simulink model "LHS_Robot"  (R2026a)
settings: Solver=FixedStepAuto  StopTime=2.72
values from neighbouring files (symbols this model uses):
  b = 4.50    (= 4.5)    [run_simulation.m]    (also in sim_dashboard.m = prs(j,2))
  c_L = 1.5813    [run_simulation.m]
  E_max = 6.6    [run_simulation.m]
  K = 0.002811691    [run_simulation.m]
  Ki = 2.5    [run_simulation.m]
  Kp = 0.18    [run_simulation.m]
  m_L = 1.1763    [run_simulation.m]
  mass = 0.85    [run_simulation.m]
  N = numel(tracks)    [route_planner.m]    (also in run_simulation.m = 48; sim_dashboard.m = size(starts, 1))
  R_wheel = 0.065/2    (= 0.0325)    [run_simulation.m]
  Ra = 7.953487304    [run_simulation.m]
  Ts = 0.02    [run_simulation.m]
  Ts_fast = 2e-5    (= 2e-05)    [run_simulation.m]
libraries: slpidlib x1
settings Model: DataDictionary=Robot.sldd  Creator=AdrianStark  LastModifiedBy=AdrianStark
settings ModelReferenceCC: ModelReferenceMinAlgLoopOccurrences=on

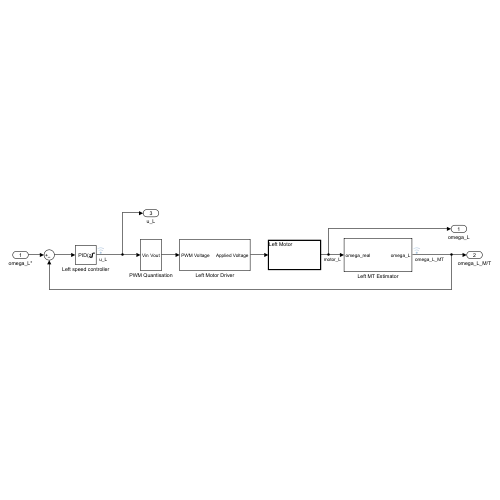
[thumbnail: Simulink's stored preview of the top-level diagram]
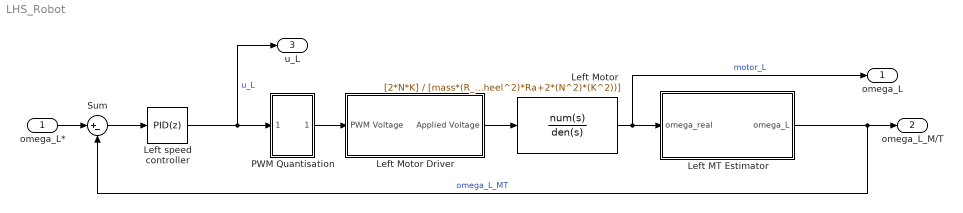
== system LHS_Robot ==
  omega_L* : Inport  OutDataTypeStr=double  PortDimensions=1  SampleTime=[0,1]
  Left MT Estimator : Subsystem
  Left Motor : TransferFcn  Numerator=[2*N*K]  Denominator=[mass*(R_wheel^2)*Ra (b*(R_wheel^2)*Ra+2*(N^2)*(K^2))]
  Left Motor Driver : Subsystem
  Left speed controller : slpidlib/PID Controller  Controller=PID  Form=Parallel  TimeDomain=Discrete-time  UseExternalTs=off  SampleTime=Ts  IntegratorMethod=Trapezoidal  FilterMethod=Forward Euler  ControllerParametersSource=internal  P=Kp  I=Ki  UseKiTs=off  D=0  UseExternalDerivativeSource=off  N=100  UseFilter=on  TunerSelectOption=Transfer Function Based (PID Tuner App)  InitialConditionSource=internal  InitialConditionForIntegrator=0  InitialConditionForFilter=0  DifferentiatorICPrevScaledInput=0  ExternalReset=none  TrackingMode=off  Kt=1  LimitOutput=on  SatLimitsSource=internal  UpperSaturationLimit=E_max  LowerSaturationLimit=0  LinearizeAsGain=on  AntiWindupMode=clamping  Kb=1  LimitIntegrator=off  UpperIntegratorSaturationLimit=inf  LowerIntegratorSaturationLimit=-inf  POutMin=[]  POutMax=[]  IOutMin=[]  IOutMax=[]  DOutMin=[]  DOutMax=[]  NOutMin=[]  NOutMax=[]  SumOutMin=[]  SumOutMax=[]  SaturationOutMin=[]  SaturationOutMax=[]  PParamMin=[]  PParamMax=[]  IParamMin=[]  IParamMax=[]  DParamMin=[]  DParamMax=[]  NParamMin=[]  NParamMax=[]  KbParamMin=[]  KbParamMax=[]  KtParamMin=[]  KtParamMax=[]  KbOutMin=[]  KbOutMax=[]  KtOutMin=[]  KtOutMax=[]  IntegratorOutMin=[]  IntegratorOutMax=[]  FilterOutMin=[]  FilterOutMax=[]  SumI1OutMin=[]  SumI1OutMax=[]  SumI2OutMin=[]  SumI2OutMax=[]  SumI3OutMin=[]  SumI3OutMax=[]  SumI4OutMin=[]  SumI4OutMax=[]  SumDOutMin=[]  SumDOutMax=[]  DifferentiatorOutMin=[]  DifferentiatorOutMax=[]  FilterDiffOutCoefMin=[]  FilterDiffOutCoefMax=[]  ReciprocalOutMin=[]  ReciprocalOutMax=[]  SumDenOutMin=[]  SumDenOutMax=[]  SumNumOutMin=[]  SumNumOutMax=[]  DivideOutMin=[]  DivideOutMax=[]  UdiffTsProdOutMin=[]  UdiffTsProdOutMax=[]  NTsProdOutMin=[]  NTsProdOutMax=[]  UintegralTsProdOutMin=[]  UintegralTsProdOutMax=[]  UngainTsProdOutMin=[]  UngainTsProdOutMax=[]  ClampingZeroOutDataTypeStr=Inherit: Inherit via back propagation  ClampingZeroOutMin=[]  ClampingZeroOutMax=[]  FilterDenConstantOutDataTypeStr=Inherit: Inherit via back propagation  FilterDenConstantOutMin=[]  FilterDenConstantOutMax=[]  PCopyOutDataTypeStr=Inherit: Inherit via back propagation  PCopyOutMin=[]  PCopyOutMax=[]  NCopyOutDataTypeStr=Inherit: Inherit via back propagation  NCopyOutMin=[]  NCopyOutMax=[]  IntegratorContinuousStateAttributes=''  IntegratorStateMustResolveToSignalObject=off  IntegratorRTWStateStorageClass=Auto  FilterContinuousStateAttributes=''  FilterStateMustResolveToSignalObject=off  FilterRTWStateStorageClass=Auto  ParallelPVariant=InternalParameters  IdealPVariant=Disabled  IVariant=InternalParameters  DVariant=InternalParameters  IntegratorVariant=Discrete  SatVariant=Enabled  AWVariant=DiscClampingParallel  PCopyVariant=Disabled  TRVariant=Disabled  FdbkBlocksVariant=Feedback  IdealPFdbkVariant=Passthrough  SatFdbkVariant=Passthrough  DerivativeFilterVariant=ForwardEulerFilter  NVariant=InternalParameters  NCopyVariant=Disabled  FilterICVariant=InternalICsFilter  IntegratorICVariant=InternalICs  ExternalResetVariant=Disabled  TRSumVariant=Passthrough  SumFdbkVariant=Enabled  SumVariant=Sum_PID  TsampFilterVariant=InternalTs  TsampNgainVariant=Passthrough  TsampIntegralVariant=Disabled_SignalSpec  ExternalSaturationOutDataTypeStr=Inherit: Same as second input  DerivativeSourceVariant=ErrorSignal  PreIntVariant=InternalPreInt
  PWM Quantisation : Subsystem
  Sum : Sum  Inputs=|+-
  omega_L : Outport
  omega_L_M/T : Outport  Port=2  OutDataTypeStr=double  PortDimensions=1  SampleTime=[0.02,0]
  u_L : Outport  Port=3
  wires:
  Left Motor/1 -> omega_L/1, Left MT Estimator/1(omega_real)  "motor_L"
  Left MT Estimator/1(omega_L) -> omega_L_M/T/1, Sum/2  "omega_L_MT"
  omega_L*/1 -> Sum/1
  Sum/1 -> Left speed controller/1
  Left speed controller/1 -> u_L/1, PWM Quantisation/1(Vin)  "u_L"
  Left Motor Driver/1(Applied Voltage) -> Left Motor/1
  PWM Quantisation/1(Vout) -> Left Motor Driver/1(PWM Voltage)

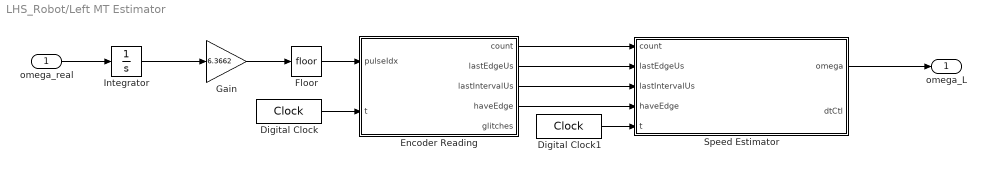
== system LHS_Robot/Left MT Estimator ==
  omega_real : Inport
  Digital Clock : DigitalClock  SampleTime=Ts_fast
  Digital Clock1 : DigitalClock  SampleTime=Ts
  Encoder Reading : MATLAB Function  TreatAsAtomicUnit=on  SystemSampleTime=Ts_fast
  Floor : Rounding
  Gain : Gain  Gain=6.3662
  Integrator : Integrator
  Speed Estimator : MATLAB Function  TreatAsAtomicUnit=on  SystemSampleTime=Ts
  omega_L : Outport
  wires:
  omega_real/1 -> Integrator/1
  Encoder Reading/3(lastIntervalUs) -> Speed Estimator/3(lastIntervalUs)
  Encoder Reading/1(count) -> Speed Estimator/1(count)
  Floor/1 -> Encoder Reading/1(pulseIdx)
  Integrator/1 -> Gain/1
  Speed Estimator/1(omega) -> omega_L/1
  Gain/1 -> Floor/1
  Encoder Reading/4(haveEdge) -> Speed Estimator/4(haveEdge)
  Digital Clock/1 -> Encoder Reading/2(t)
  Encoder Reading/2(lastEdgeUs) -> Speed Estimator/2(lastEdgeUs)
  Digital Clock1/1 -> Speed Estimator/5(t)

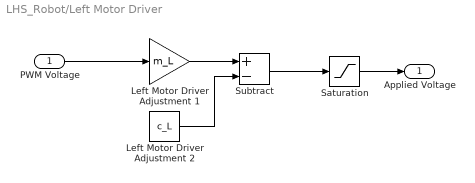
== system LHS_Robot/Left Motor Driver ==
  PWM Voltage : Inport
  Left Motor Driver Adjustment 1 : Gain  Gain=m_L
  Left Motor Driver Adjustment 2 : Constant  Value=c_L
  Saturation : Saturate  UpperLimit=6.6  LowerLimit=0
  Subtract : Sum  Inputs=+-
  Applied Voltage : Outport
  wires:
  Saturation/1 -> Applied Voltage/1
  Left Motor Driver Adjustment 2/1 -> Subtract/2
  PWM Voltage/1 -> Left Motor Driver Adjustment 1/1
  Subtract/1 -> Saturation/1
  Left Motor Driver Adjustment 1/1 -> Subtract/1

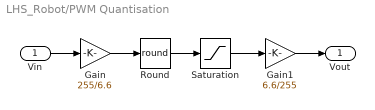
== system LHS_Robot/PWM Quantisation ==
  Vin : Inport
  Gain : Gain  Gain=255/6.6
  Gain1 : Gain  Gain=6.6/255
  Round : Rounding  Operator=round
  Saturation : Saturate  UpperLimit=255  LowerLimit=0
  Vout : Outport
  wires:
  Gain1/1 -> Vout/1
  Vin/1 -> Gain/1
  Saturation/1 -> Gain1/1
  Round/1 -> Saturation/1
  Gain/1 -> Round/1

== matlab function LHS_Robot/Left MT Estimator/Speed Estimator ==
  data: count input; lastEdgeUs input; lastIntervalUs input; haveEdge input; omega output; t input; dtCtl output
function [omega, dtCtl] = mtTickEstimator(count, lastEdgeUs, lastIntervalUs, haveEdge, t)
%MTTICKESTIMATOR  Simulink model of the per-tick estimator in loop().
%
%   One instance per wheel. MATLAB Function block, Sample time = 0.020
%   (TICK_MS). Inputs come from encoderISR through a Rate Transition.
%
%   Reproduces, in order:
%     1. the ring buffer snapshot of (count, lastEdgeUs)
%     2. M/T over the LONGEST valid span, not just the full gate
%     3. the T fallback (one interval, reciprocated, decaying as 1/t)
%     4. the staleness ceiling and the stall timeout
%     5. the measured, clamped dt handed to the PID
%
%   dtCtl is constant at 0.020 in simulation because the model has no
%   serial writes to delay a tick. Leave the clamp in anyway - it costs
%   nothing and it documents what the firmware does.

%#codegen

% ---- Constants, matching the sketch -----------------------------------
WINDOW_TICKS     = 3;
NRING            = WINDOW_TICKS + 1;             % 4 slots, 60 ms max span
PULSES_PER_REV   = 40;                           % 20 slots x 2 edges x gear 1.0
RAD_PER_PULSE    = 2*pi/PULSES_PER_REV;          % 0.157080 rad
STALL_TIMEOUT_US = uint32(500000);
TICK_MS          = 20;
DT_MIN_S         = TICK_MS*0.0005;               % 0.010 s
DT_MAX_S         = TICK_MS*0.0040;               % 0.080 s

persistent ringCount ringEdge head fill lastCtlUs ctlPrimed
if isempty(head)
    ringCount = zeros(1, NRING, 'uint32');
    ringEdge  = zeros(1, NRING, 'uint32');
    head      = 0;                               % 0-based, as in C
    fill      = 0;
    lastCtlUs = uint32(0);
    ctlPrimed = false;
end

nowUs = uint32(t*1e6);

% ---- Snapshot into the ring -------------------------------------------
head = mod(head + 1, NRING);
ringCount(head+1) = count;
ringEdge(head+1)  = lastEdgeUs;
if fill <= WINDOW_TICKS
    fill = fill + 1;
end

omega  = 0;
haveMT = false;

% ---- M/T over the longest valid span ----------------------------------
% Search from the OLDEST usable snapshot forward, break on the first hit,
% so the span grows as history accumulates rather than jumping when the
% gate fills.
if fill >= 2
    startBack = fill - 1;
else
    startBack = 0;
end

for back = startBack:-1:1
    idx = mod(head + NRING - back, NRING);       % 0-based, as in C
    if ringCount(idx+1) < 1
        continue                                  % no edge existed yet
    end
    if count <= ringCount(idx+1)
        continue                                  % no new pulse since
    end
    dtEdgeUs = lastEdgeUs - ringEdge(idx+1);
    if dtEdgeUs == 0
        continue
    end
    omega  = double(count - ringCount(idx+1)) * RAD_PER_PULSE * 1e6 / double(dtEdgeUs);
    haveMT = true;
    break
end

% ---- T fallback --------------------------------------------------------
if ~haveMT && haveEdge && lastIntervalUs > 0
    sinceUs = nowUs - lastEdgeUs;
    if sinceUs < STALL_TIMEOUT_US
        if sinceUs > lastIntervalUs
            effUs = sinceUs;
        else
            effUs = lastIntervalUs;
        end
        omega = RAD_PER_PULSE * 1e6 / double(effUs);
    end
end

% ---- Staleness ceiling -------------------------------------------------
% The M/T window ends at the LAST EDGE, not at now, so without this a
% stopped wheel keeps re-reporting the speed from before it stopped.
if haveEdge
    sinceUs = nowUs - lastEdgeUs;
    if sinceUs >= STALL_TIMEOUT_US
        omega = 0;
    elseif sinceUs > 0
        bound = RAD_PER_PULSE * 1e6 / double(sinceUs);
        if omega > bound
            omega = bound;
        end
    end
end

% ---- Measured control interval ----------------------------------------
dtCtl = TICK_MS/1000;
if ctlPrimed
    dtCtl = double(nowUs - lastCtlUs) * 1e-6;
end
ctlPrimed = true;
lastCtlUs = nowUs;
if dtCtl < DT_MIN_S
    dtCtl = DT_MIN_S;
end
if dtCtl > DT_MAX_S
    dtCtl = DT_MAX_S;
end
end

== matlab function LHS_Robot/Left MT Estimator/Encoder Reading ==
  data: pulseIdx input; count output; t input; lastEdgeUs output; lastIntervalUs output; haveEdge output; glitches output
function [count, lastEdgeUs, lastIntervalUs, haveEdge, glitches] = encoderISR(pulseIdx, t)
%ENCODERISR  Simulink model of edgeSeen() in DualWheelDriveBT.ino.
%
%   Put this in a MATLAB Function block running at the FAST rate
%   (Sample time = 4e-6 to match micros(), or 1e-5 if you can live with
%   coarser edge timestamps).
%
%   pulseIdx : floor(theta / RAD_PER_PULSE) from the continuous plant
%   t        : simulation time [s], from a Digital Clock at this rate
%
%   Outputs mirror g_count, g_lastEdgeUs, g_lastIntervalUs, g_haveEdge.
%   glitches is a diagnostic with no firmware equivalent in the snapshot;
%   if it climbs during a run your fast step is too coarse or your plant
%   is producing edges the real disc could not.
 
%#codegen
 
% ---- Constants, derived exactly as the sketch derives them -------------
%   SLOT_PERIOD_MIN_US = 1e6 / (W_COMMAND_MAX/2pi * PULSES_PER_WHEEL_REV)
%                      = 1e6 / (60/2pi * 40) = 2618.0 us
%   MIN_PULSE_US       = 2618.0 * SLOT_DUTY_MIN(0.10) * MIN_PULSE_FRACTION(0.25)
%                      = 65.45 -> 65 (uint32 truncation in C)
MIN_PULSE_US  = uint32(65);
 
persistent cnt lastEdge lastIvl have prevIdx glitch
if isempty(cnt)
    cnt     = uint32(0);
    lastEdge= uint32(0);
    lastIvl = uint32(0);
    have    = false;
    prevIdx = pulseIdx;
    glitch  = uint32(0);
end
 
% micros(): free running, 4 us granularity. Rollover at 71.6 min is NOT
% modelled - MATLAB's uint32 saturates where C wraps. Keep runs short.
nowUs = uint32(t*1e6);
 
if pulseIdx ~= prevIdx
    if pulseIdx - prevIdx > 1 || prevIdx - pulseIdx > 1
        glitch = glitch + uint32(1);   % more than one edge per step: step too coarse
    end
    prevIdx = pulseIdx;
 
    if have && (nowUs - lastEdge) < MIN_PULSE_US
        % Rejected as a glitch. No count, no timestamp update - exactly
        % as the ISR does, which is why a rejected edge is invisible to
        % the estimator rather than being a short interval.
        glitch = glitch + uint32(1);
    else
        if have
            lastIvl = nowUs - lastEdge;
        else
            lastIvl = uint32(0);
        end
        lastEdge = nowUs;
        have     = true;
        cnt      = cnt + uint32(1);
    end
end
 
count          = cnt;
lastEdgeUs     = lastEdge;
lastIntervalUs = lastIvl;
haveEdge       = have;
glitches       = glitch;
end
